simulink model "pmsm_model"  (R2021a)
settings: Solver=ode15s  StartTime=0.0  StopTime=1  RelTol=1e-3
undefined symbols (not defined in the file or in its folder): P
libraries: fl_lib x5, nesl_utility x4, spsVoltageMeasurementLib x3, ee_lib x3, spsGroundLib x2, mcbcontrolslib x2, spsThreePhaseProgrammableVoltageSourceLib x1, spspowerguiLib x1
settings Model: Creator=AHMED  LastModifiedBy=AHMED

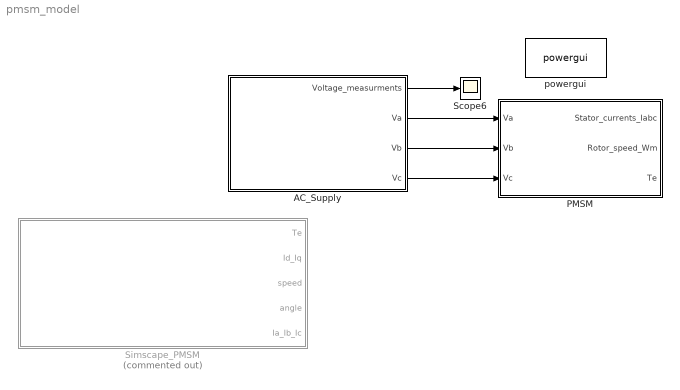
== system pmsm_model ==
  AC_Supply : Subsystem  mask{V_rms=380}
  PMSM : Subsystem  mask{Ld=0.0057, Lq=0.0125, lamda_pm=0.123, R=1.2, P=4, J=0.0001, b=0}
  Scope6 : Scope
  Simscape_PMSM : Subsystem  Commented=on
  powergui : spspowerguiLib/powergui  Priority=1  SimulationMode=Continuous  SampleTime=50e-6  frequency=60  Iterations=50  frequencyindice=60  Pbase=100e6  ErrMax=1e-4  UnitsV=kV  UnitsW=MW  buscounter=0  FunctionMessages=off  echomessages=off  EnableUseOfTLC=off  CurrentSourceSwitches=off  DisableSnubberDevices=off  DisableRonSwitches=off  DisableVfSwitches=off  DisplayEquations=off  AutomaticDiscreteSolvers=off  SolverType=Tustin/Backward Euler (TBE)  Interpol=off  ExternalGateDelay=off  methode=off  Ts=100  x0status=blocks  SPID=on  SwTol=0  HookPort=off  NonlinearTolerance=1e-4  nMaxIteration=100  ContinueOnMaxIteration=off  RestoreLinks=warning  ResistiveCurrentMeasurement=off  Frange=[0:2:500]  Ylog=off  Xlog=on  ShowGrid=off  save=off  variable=ZData  structure=0  ZoomFFT=off  StartTime=0.0  cycles=1  DisplayStyle=1  fundamental=60  FreqAxis=off  MaxFrequency=1000  frequencyindicesteady=1  RmsSteady=1  display=off
  wires:
  AC_Supply/2(Va) -> PMSM/1(Va)
  AC_Supply/3(Vb) -> PMSM/2(Vb)
  AC_Supply/4(Vc) -> PMSM/3(Vc)
  AC_Supply/1(Voltage_measurments) -> Scope6/1

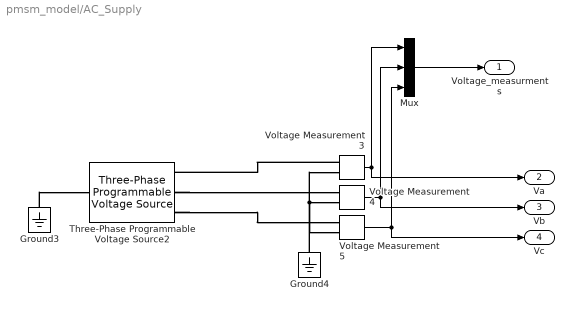
== system pmsm_model/AC_Supply ==
  Ground3 : spsGroundLib/Ground  LConnTagsString=a
  Ground4 : spsGroundLib/Ground  LConnTagsString=a
  Mux : Mux  Inputs=3
  Three-Phase Programmable Voltage Source2 : spsThreePhaseProgrammableVoltageSourceLib/Three-Phase Programmable Voltage Source  PositiveSequence=[V_rms 0 60]  VariationEntity=None  VariationType=Table of time-amplitude pairs  VariationTypeAlt=Step  VariationStep=0.5  VariationRate=10  VariationMagnitude=0.3  VariationFrequency=2  VariationTiming=[1 2]  VariationPhaseA=off  Amplitudes=[1 0.8 1.2 1.0]  TimeValues=[0 0.1 0.15 0.2]  HarmonicGeneration=off  HarmonicA=[3 0.2 -25 0]  HarmonicB=[2 0.15 35 2]  Timing="[0.05  3]"  BusType=swing  Pref=0  Qref=0  Qmin=-inf  Qmax=inf
  Voltage Measurement3 : spsVoltageMeasurementLib/Voltage Measurement  PhasorSimulation=off  OutputType=Complex  PSBequivalent=0
  Voltage Measurement4 : spsVoltageMeasurementLib/Voltage Measurement  PhasorSimulation=off  OutputType=Complex  PSBequivalent=0
  Voltage Measurement5 : spsVoltageMeasurementLib/Voltage Measurement  PhasorSimulation=off  OutputType=Complex  PSBequivalent=0
  Voltage_measurments : Outport
  Va : Outport  Port=2
  Vb : Outport  Port=3
  Vc : Outport  Port=4
  wires:
  Voltage Measurement3/1 -> Va/1, Mux/1
  Voltage Measurement4/1 -> Vb/1, Mux/2
  Voltage Measurement5/1 -> Vc/1, Mux/3
  Mux/1 -> Voltage_measurments/1
  connections:
  Voltage Measurement3/LConn1 -- Three-Phase Programmable Voltage Source2/RConn1
  Ground4/LConn1 -- Voltage Measurement5/LConn2 -- Voltage Measurement3/LConn2 -- Voltage Measurement4/LConn2
  Three-Phase Programmable Voltage Source2/RConn3 -- Voltage Measurement5/LConn1
  Three-Phase Programmable Voltage Source2/RConn2 -- Voltage Measurement4/LConn1
  Ground3/LConn1 -- Three-Phase Programmable Voltage Source2/LConn1

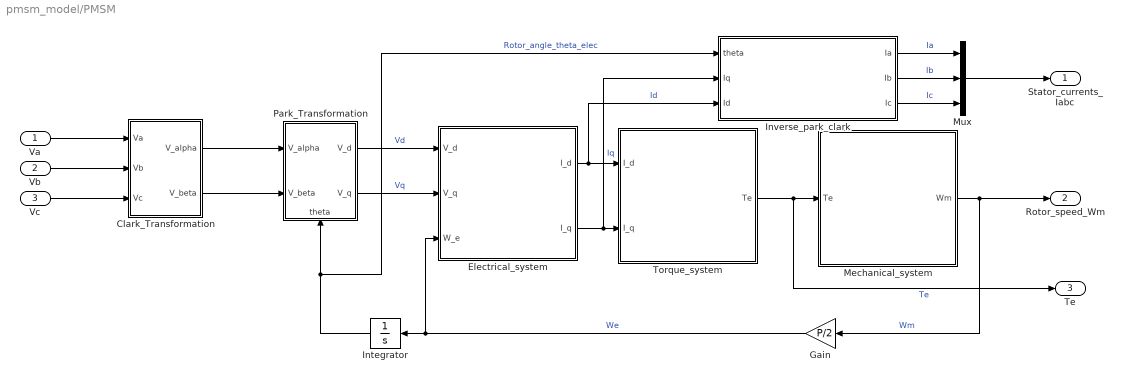
== system pmsm_model/PMSM ==
  Va : Inport
  Vb : Inport  Port=2
  Vc : Inport  Port=3
  Clark_Transformation : Subsystem
  Electrical_system : Subsystem
  Gain : Gain  Gain=P/2
  Integrator : Integrator
  Inverse_park_clark : Subsystem
  Mechanical_system : Subsystem
  Mux : Mux  Inputs=3
  Park_Transformation : Subsystem
      settings: PortSchema="{\"entries\":[{\"content\":{\"sides\":[{\"content\":{\"connectorIds\":[\"In1\",\"In2\"]},\"type\":\"ConnectorPlacement.EquallySpacedRectSide\",\"uuid\":\"a5303260-9056-4ba9-bf21-9d9e68c76aad\"},{\"content\":{\"connectorIds\":[\"Out1\",\"Out2\"],\"side\":\"RIGHT\"},\"type\":\"ConnectorPlacement.EquallySpacedRectSide\",\"uuid\":\"bf8eba39-f781-4672-b99d-9d1cb4b6396f\"},{\"content\":{\"connectorIds\":[],\"side\":\"TOP\"},\"type\":\"ConnectorPlacement.EquallySpacedRectSide\",\"uuid\":\"4985423e-053d-4914-82fe-b9dd9f427f0d\"},{\"content\":{\"connectorIds\":[\"In3\"],\"side\":\"BOTTOM\"},\"type\":\"ConnectorPlacement.EquallySpacedRectSide\",\"uuid\":\"0752c2be-c5bb-44b3-a6b0-4f5b66c2ccb1\"}]},\"type\":\"ConnectorPlacement.EquallySpacedConnector\",\"uuid\":\"0aeb7acd-9c9e-4bf3-9d65-4f157eb3bd0a\"}],\"packageUris\":[\"http://schema.mathworks.com/mf0/Connector/R2020b\"],\"version\":\"1.0\"}"
  Torque_system : Subsystem
  Stator_currents_Iabc : Outport
  Rotor_speed_Wm : Outport  Port=2
  Te : Outport  Port=3
  wires:
  Va/1 -> Clark_Transformation/1(Va)
  Vb/1 -> Clark_Transformation/2(Vb)
  Vc/1 -> Clark_Transformation/3(Vc)
  Clark_Transformation/1(V_alpha) -> Park_Transformation/1(V_alpha)
  Clark_Transformation/2(V_beta) -> Park_Transformation/2(V_beta)
  Park_Transformation/1(V_d) -> Electrical_system/1(V_d)  "Vd"
  Park_Transformation/2(V_q) -> Electrical_system/2(V_q)  "Vq"
  Electrical_system/1(I_d) -> Torque_system/1(I_d), Inverse_park_clark/3(Id)  "Id"
  Electrical_system/2(I_q) -> Inverse_park_clark/2(Iq), Torque_system/2(I_q)  "Iq"
  Torque_system/1(Te) -> Te/1, Mechanical_system/1(Te)  "Te"
  Mechanical_system/1(Wm) -> Gain/1, Rotor_speed_Wm/1  "Wm"
  Gain/1 -> Integrator/1, Electrical_system/3(W_e)  "We"
  Integrator/1 -> Inverse_park_clark/1(theta), Park_Transformation/3(theta)  "Rotor_angle_theta_elec"
  Inverse_park_clark/1(Ia) -> Mux/1  "Ia"
  Inverse_park_clark/2(Ib) -> Mux/2  "Ib"
  Inverse_park_clark/3(Ic) -> Mux/3  "Ic"
  Mux/1 -> Stator_currents_Iabc/1

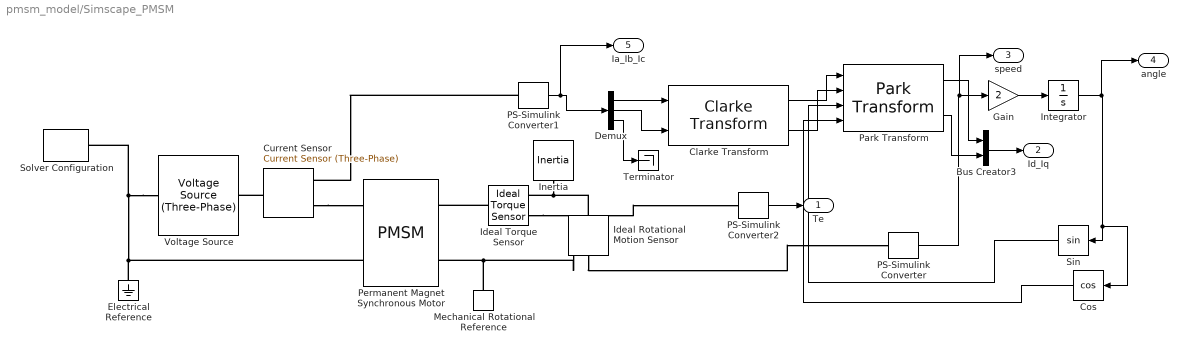
== system pmsm_model/Simscape_PMSM ==
  Bus Creator3 : BusCreator  Inputs=2
  Clarke Transform : mcbcontrolslib/Clarke Transform  VariantControl=Variant2
  Cos : Trigonometry  Operator=cos
  Current Sensor : ee_lib/Sensors & Transducers/Current Sensor (Three-Phase)
  Demux : Demux  Outputs=3
  Electrical Reference : fl_lib/Electrical/Electrical Elements/Electrical Reference
  Gain : Gain  Gain=2
  Ideal Rotational Motion Sensor : fl_lib/Mechanical/Mechanical Sensors/Ideal Rotational Motion Sensor  wrap_angle=simscape.enum.onoff.off  offset=0 deg
      settings: SourceProductName=Foundation Library
  Ideal Torque Sensor : fl_lib/Mechanical/Mechanical Sensors/Ideal Torque Sensor
      settings: SourceProductName=Foundation Library
  Inertia : fl_lib/Mechanical/Rotational Elements/Inertia  inertia="0.0001  kg*m^2"  num_ports=foundation.enum.numPorts2.one  w_specify=off  w_priority=High  w=0 rad/s  w_nominal_specify=off  w_nominal_unit=rad/s  w_nominal_value=1  t_specify=off  t_priority=None  t=0 N*m  t_nominal_specify=off  t_nominal_unit=N*m  t_nominal_value=1
  Integrator : Integrator
  Mechanical Rotational Reference : fl_lib/Mechanical/Rotational Elements/Mechanical Rotational Reference
  PS-Simulink Converter : nesl_utility/PS-Simulink Converter  PhysicalDomain=network_engine_domain  SubClassName=ps_output  LeftPortType=input  RightPortType=output  PseudoPeriodic=off  Frequencies=[]  Unit=rad/s  AffineConversion=off
      settings: SourceProductBaseCode=PW,SS
  PS-Simulink Converter1 : nesl_utility/PS-Simulink Converter  PhysicalDomain=network_engine_domain  SubClassName=ps_output  LeftPortType=input  RightPortType=output  PseudoPeriodic=off  Frequencies=[]  Unit=A  AffineConversion=off
      settings: SourceProductBaseCode=PW,SS
  PS-Simulink Converter2 : nesl_utility/PS-Simulink Converter  PhysicalDomain=network_engine_domain  SubClassName=ps_output  LeftPortType=input  RightPortType=output  PseudoPeriodic=off  Frequencies=[]  Unit=N*m  AffineConversion=off
      settings: SourceProductBaseCode=PW,SS
  Park Transform : mcbcontrolslib/Park Transform  AxisAlignment=D-axis
      settings: SourceProductBaseCode=MT
  Permanent Magnet Synchronous Motor : ee_lib/Electromechanical/Permanent Magnet/PMSM  winding_type=ee.enum.statorconnection.wye  machine_param=ee.enum.pmsm.parameterization.constant  nPolePairs=P/2  pmflux_param=1  pm_flux_linkage=PM Wb  torque_constant=0.18 N*m/A  back_emf_constant=0.18 V/(rad/s)  stator_param=1  Ld=Ld H  Lq=Lq H  idVec=[-200, 0, 200] A  iqVec=[-200, 0, 200] A  LdMatrix=0.0002 * ones(3, 3) H  LqMatrix=0.0002 * ones(3, 3) H  PmMatrix=0.1 * ones(3, 3) Wb  ktMatrix=0.18 * ones(3, 3) N*m/A  keMatrix=0.18 * ones(3, 3) V/(rad/s)  L0=0 H  Ls=0.0002 H  Lm=-0.00002 H  Ms=0.00002 H  Rs=r Ohm  zero_sequence=ee.enum.park.zerosequence.include  J=0 kg*m^2  lam=0 N*m/(rad/s)  axes_param=2  i_d_specify=off  i_d_priority=None  i_d=0 A  i_d_nominal_specify=off  i_d_nominal_unit=A  i_d_nominal_value=1  i_q_specify=off  i_q_priority=None  i_q=0 A  i_q_nominal_specify=off  i_q_nominal_unit=A  i_q_nominal_value=1  torque_specify=off  torque_priority=None  torque=0 N*m  torque_nominal_specify=off  torque_nominal_unit=N*m  torque_nominal_value=1  angular_velocity_specify=on  angular_velocity_priority=None  angular_velocity=0 rpm  angular_velocity_nominal_specify=off  angular_velocity_nominal_unit=rpm  angular_velocity_nominal_value=1  angular_position_specify=on  angular_position_priority=High  angular_position=0 deg  angular_position_nominal_specify=off  angular_position_nominal_unit=deg  angular_position_nominal_value=1  loss_param=ee.enum.ironloss.none  losses_oc=[0, 0, 0] W  losses_sc=[0, 0, 0] W  f_losses=60 Hz  Isc_losses=95 A  Tmeas=298.15 K  alpha=3.93e-3 1/K  alpha_flux=-0.001 1/K  stator_thermal_mass=100 J/K  rotor_thermal_mass=200 J/K  Rm_percent_rotor=90  Rd_percent_rotor=30  temperatureA_specify=off  temperatureA_priority=High  temperatureA=25 degC  temperatureA_nominal_specify=off  temperatureA_nominal_unit=degC  temperatureA_nominal_value=1  temperatureB_specify=off  temperatureB_priority=High  temperatureB=25 degC  temperatureB_nominal_specify=off  temperatureB_nominal_unit=degC  temperatureB_nominal_value=1  temperatureC_specify=off  temperatureC_priority=High  temperatureC=25 degC  temperatureC_nominal_specify=off  temperatureC_nominal_unit=degC  temperatureC_nominal_value=1  temperatureR_specify=off  temperatureR_priority=High  temperatureR=25 degC  temperatureR_nominal_specify=off  temperatureR_nominal_unit=degC  temperatureR_nominal_value=1
      settings: InternalSimscapePortConfiguration="{\"Bottom\":[],\"Left\":[{\"id\":\"N\",\"label\":\"~\",\"type\":\"foundation.electrical.three_phase\"},{\"id\":\"n\",\"label\":\"n\",\"type\":\"foundation.electrical.electrical\"}],\"Right\":[{\"id\":\"R\",\"label\":\"R\",\"type\":\"foundation.mechanical.rotational.rotational\"},{\"id\":\"C\",\"label\":\"C\",\"type\":\"foundation.mechanical.rotational.rotational\"}],\"Top\":[]}"
  Sin : Trigonometry
  Solver Configuration : nesl_utility/Solver Configuration  PhysicalDomain=network_engine_domain  SubClassName=solver  LeftPortType=input  RightPortType=generic  Tones=[]  Harmonics=[]  SimulateNoise=off  Profile=off  UseLocalSampling=off  EnableSwitchedLinearOptims=on  FrequencyDomain=off  UseCCode=off  RelTol=0.001  AbsTol=1e-06  MinStep=1e-09  ToWorkspace=off  RevertToSquareIcSolve=off  NumHomotopyIterations=100  PhasorMode=off  PhasorModeNumHarmonics=1  DoDC=off  ResidualTolerance=1e-09  UseLocalSolver=off  LocalSolverChoice=NE_BACKWARD_EULER_ADVANCER  LocalSolverSampleTime=0.001  DoFixedCost=off  MaxNonlinIter=3  MaxModeIter=2  ComputeImpulses=off  ImpulseIterations=2  LinearAlgebra=auto  EquationFormulation=NE_TIME_EF  DelaysMemoryBudget=1024  AutomaticFiltering=on  FilteringTimeConstant=0.001  PartitionStorageMethod=AS_NEEDED  PartitionMemoryBudget=1024  PartitionMethod=ROBUST
      settings: SourceProductBaseCode=PW,SS
  Terminator : Terminator
  Voltage Source : ee_lib/Sources/Voltage Source (Three-Phase)  vline_rms=380 V  shift=0 deg  freq=60 Hz  impedance_option=0  SShortCircuit=1e6 V*A  XR=15  R=0.01 Ohm  L=3.97e-4 H  G_parasitic=0 1/Ohm  harmonic_option=0  harmonic_orders=[5, 7, 11, 13]  harmonic_ratios=[.1, .1, .1, .1]  I_specify=off  I_priority=None  I=[ 0 0 0 ] A  I_nominal_specify=off  I_nominal_unit=A  I_nominal_value=1
      settings: SourceProductBaseCode=PS
  Te : Outport
  Id_Iq : Outport  Port=2
  speed : Outport  Port=3
  angle : Outport  Port=4
  Ia_Ib_Ic : Outport  Port=5
  wires:
  Integrator/1 -> angle/1, Cos/1, Sin/1
  Sin/1 -> Park Transform/3
  Cos/1 -> Park Transform/4
  Gain/1 -> Integrator/1
  Demux/2 -> Clarke Transform/2
  PS-Simulink Converter/1 -> speed/1, Gain/1
  Clarke Transform/2 -> Park Transform/2
  Bus Creator3/1 -> Id_Iq/1
  PS-Simulink Converter1/1 -> Ia_Ib_Ic/1, Demux/1
  Park Transform/2 -> Bus Creator3/2
  Demux/1 -> Clarke Transform/1
  Clarke Transform/1 -> Park Transform/1
  Park Transform/1 -> Bus Creator3/1
  Demux/3 -> Terminator/1
  PS-Simulink Converter2/1 -> Te/1
  connections:
  Inertia/LConn1 -- Ideal Rotational Motion Sensor/LConn1 -- Ideal Torque Sensor/RConn1
  Ideal Torque Sensor/LConn1 -- Permanent Magnet Synchronous Motor/RConn1
  Permanent Magnet Synchronous Motor/RConn2 -- Ideal Rotational Motion Sensor/RConn1 -- Mechanical Rotational Reference/LConn1
  Current Sensor/RConn2 -- Permanent Magnet Synchronous Motor/LConn1
  Ideal Torque Sensor/RConn2 -- PS-Simulink Converter2/LConn1
  Voltage Source/LConn1 -- Solver Configuration/RConn1 -- Electrical Reference/LConn1 -- Permanent Magnet Synchronous Motor/LConn2
  PS-Simulink Converter1/LConn1 -- Current Sensor/RConn1
  Ideal Rotational Motion Sensor/RConn2 -- PS-Simulink Converter/LConn1
  Current Sensor/LConn1 -- Voltage Source/RConn1

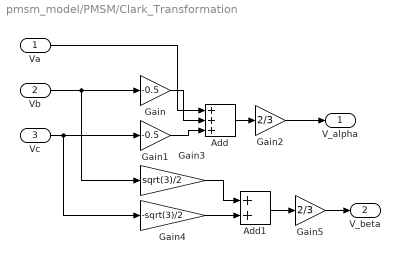
== system pmsm_model/PMSM/Clark_Transformation ==
  Va : Inport
  Vb : Inport  Port=2
  Vc : Inport  Port=3
  Add : Sum  Inputs=+++
  Add1 : Sum
  Gain : Gain  Gain=-0.5
  Gain1 : Gain  Gain=-0.5
  Gain2 : Gain  Gain=2/3
  Gain3 : Gain  Gain=sqrt(3)/2
  Gain4 : Gain  Gain=-sqrt(3)/2
  Gain5 : Gain  Gain=2/3
  V_alpha : Outport
  V_beta : Outport  Port=2
  wires:
  Vb/1 -> Gain3/1, Gain/1
  Vc/1 -> Gain4/1, Gain1/1
  Gain/1 -> Add/2
  Gain1/1 -> Add/3
  Va/1 -> Add/1
  Add/1 -> Gain2/1
  Gain2/1 -> V_alpha/1
  Gain4/1 -> Add1/2
  Gain3/1 -> Add1/1
  Add1/1 -> Gain5/1
  Gain5/1 -> V_beta/1

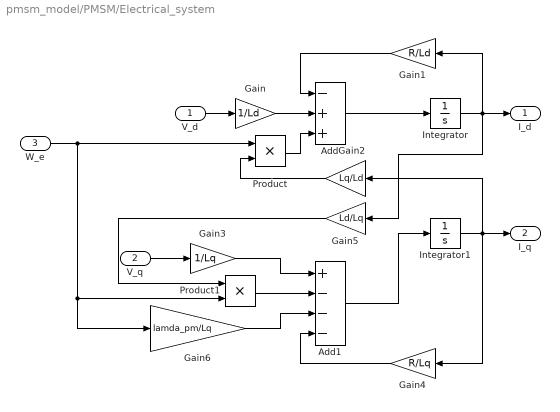
== system pmsm_model/PMSM/Electrical_system ==
  V_d : Inport
  V_q : Inport  Port=2
  W_e : Inport  Port=3
  Add : Sum  Inputs=-++
  Add1 : Sum  Inputs=+---
  Gain : Gain  Gain=1/Ld
  Gain1 : Gain  Gain=R/Ld
  Gain2 : Gain  Gain=Lq/Ld
  Gain3 : Gain  Gain=1/Lq
  Gain4 : Gain  Gain=R/Lq
  Gain5 : Gain  Gain=Ld/Lq
  Gain6 : Gain  Gain=lamda_pm/Lq
  Integrator : Integrator
  Integrator1 : Integrator
  Product : Product
  Product1 : Product
  I_d : Outport
  I_q : Outport  Port=2
  wires:
  Integrator/1 -> Gain5/1, Gain1/1, I_d/1
  Integrator1/1 -> Gain4/1, Gain2/1, I_q/1
  V_d/1 -> Gain/1
  Gain/1 -> Add/2
  Gain1/1 -> Add/1
  Add/1 -> Integrator/1
  Gain2/1 -> Product/2
  W_e/1 -> Gain6/1, Product1/2, Product/1
  Product/1 -> Add/3
  V_q/1 -> Gain3/1
  Gain3/1 -> Add1/1
  Gain4/1 -> Add1/4
  Gain5/1 -> Product1/1
  Product1/1 -> Add1/2
  Gain6/1 -> Add1/3
  Add1/1 -> Integrator1/1

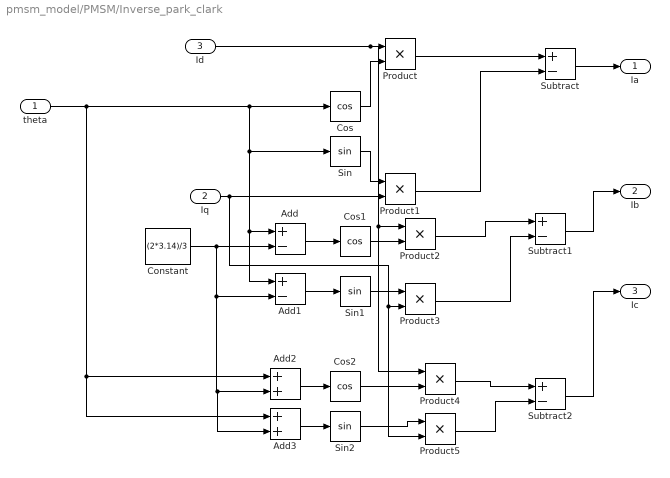
== system pmsm_model/PMSM/Inverse_park_clark ==
  theta : Inport
  Iq : Inport  Port=2
  Id : Inport  Port=3
  Add : Sum  Inputs=+-
  Add1 : Sum  Inputs=+-
  Add2 : Sum
  Add3 : Sum
  Constant : Constant  Value=(2*3.14)/3
  Cos : Trigonometry  Operator=cos
  Cos1 : Trigonometry  Operator=cos
  Cos2 : Trigonometry  Operator=cos
  Product{,1..5} (6 alike) : Product
  Sin : Trigonometry
  Sin1 : Trigonometry
  Sin2 : Trigonometry
  Subtract : Sum  Inputs=+-
  Subtract1 : Sum  Inputs=+-
  Subtract2 : Sum  Inputs=+-
  Ia : Outport
  Ib : Outport  Port=2
  Ic : Outport  Port=3
  wires:
  Subtract/1 -> Ia/1
  theta/1 -> Add3/1, Add2/1, Cos/1, Add1/1, Add/1, Sin/1
  Id/1 -> Product4/1, Product2/1, Product/1
  Cos/1 -> Product/2
  Product/1 -> Subtract/1
  Iq/1 -> Product5/2, Product3/2, Product1/2
  Sin/1 -> Product1/1
  Product1/1 -> Subtract/2
  Add/1 -> Cos1/1
  Add1/1 -> Sin1/1
  Cos1/1 -> Product2/2
  Sin1/1 -> Product3/1
  Product2/1 -> Subtract1/1
  Product3/1 -> Subtract1/2
  Subtract1/1 -> Ib/1
  Constant/1 -> Add3/2, Add2/2, Add1/2, Add/2
  Subtract2/1 -> Ic/1
  Product4/1 -> Subtract2/1
  Product5/1 -> Subtract2/2
  Cos2/1 -> Product4/2
  Sin2/1 -> Product5/1
  Add2/1 -> Cos2/1
  Add3/1 -> Sin2/1

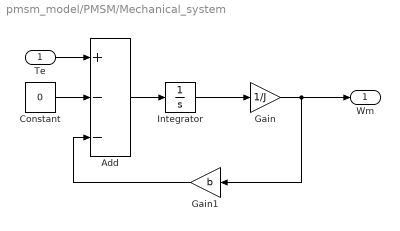
== system pmsm_model/PMSM/Mechanical_system ==
  Te : Inport
  Add : Sum  Inputs=+--
  Constant : Constant  Value=0
  Gain : Gain  Gain=1/J
  Gain1 : Gain  Gain=b
  Integrator : Integrator
  Wm : Outport
  wires:
  Gain/1 -> Wm/1, Gain1/1
  Te/1 -> Add/1
  Constant/1 -> Add/2
  Gain1/1 -> Add/3
  Add/1 -> Integrator/1
  Integrator/1 -> Gain/1

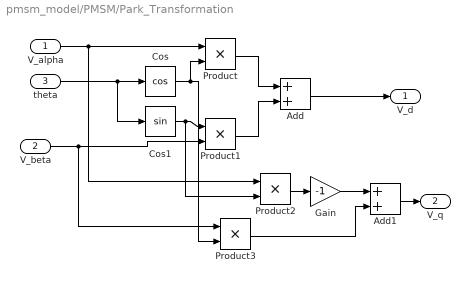
== system pmsm_model/PMSM/Park_Transformation ==
  V_alpha : Inport
  V_beta : Inport  Port=2
  theta : Inport  Port=3
  Add : Sum
  Add1 : Sum
  Cos : Trigonometry  Operator=cos
  Cos1 : Trigonometry
  Gain : Gain  Gain=-1
  Product{,1..3} (4 alike) : Product
  V_d : Outport
  V_q : Outport  Port=2
  wires:
  theta/1 -> Cos1/1, Cos/1
  V_alpha/1 -> Product2/1, Product/1
  Cos/1 -> Product3/2, Product/2
  Cos1/1 -> Product2/2, Product1/1
  V_beta/1 -> Product3/1, Product1/2
  Product/1 -> Add/1
  Product1/1 -> Add/2
  Add/1 -> V_d/1
  Product2/1 -> Gain/1
  Gain/1 -> Add1/1
  Product3/1 -> Add1/2
  Add1/1 -> V_q/1

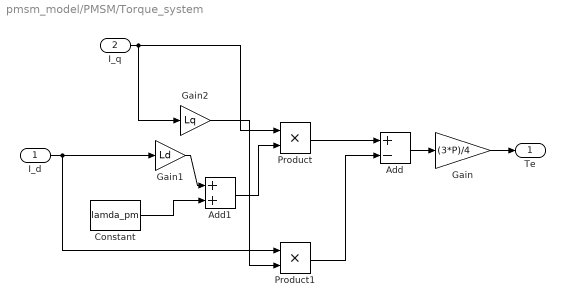
== system pmsm_model/PMSM/Torque_system ==
  I_d : Inport
  I_q : Inport  Port=2
  Add : Sum  Inputs=+-
  Add1 : Sum
  Constant : Constant  Value=lamda_pm
  Gain : Gain  Gain=(3*P)/4
  Gain1 : Gain  Gain=Ld
  Gain2 : Gain  Gain=Lq
  Product : Product
  Product1 : Product
  Te : Outport
  wires:
  Add/1 -> Gain/1
  Gain/1 -> Te/1
  I_d/1 -> Product1/1, Gain1/1
  Constant/1 -> Add1/2
  Gain1/1 -> Add1/1
  Add1/1 -> Product/2
  I_q/1 -> Gain2/1, Product/1
  Product/1 -> Add/1
  Gain2/1 -> Product1/2
  Product1/1 -> Add/2
